simulink library "sm_wheel_loader_lib"  (R2025a)
settings: Solver=VariableStepAuto  StartTime=0.0  StopTime=10.0  RelTol=1e-3
undefined symbols (not defined in the file): AToTOrificeVector, BiPOrificeVector, boomHEArea, boomREArea, BToTOrificeVector, fluids, GRake, GToothL, GToothR, HMPST, HydFcnParams, logLoad, Position, PToAOrificeVector, PToBOrificeVector, RakeL, RakeR, testInput, Wheel_Loader, X, Y, Z
libraries: sm_lib x694, fl_lib x183, nesl_utility x74, SimscapeFluids_lib x62, sdl_lib x25, cvt_components_lib x25, simulink_extras x5, $bdroot x4, wheel_loader_contact_lib x4, ee_lib x2, SignalEditorBlockLib x1, batteryecm_lib x1
(part 1 of 26)
Description:
  | Copyright 2023-2025 The MathWorks, Inc.
settings Model: VariantFading=off  Creator=smiller  LastModifiedBy=smiller
settings RTWCC: GPUComputeCapability=3.5

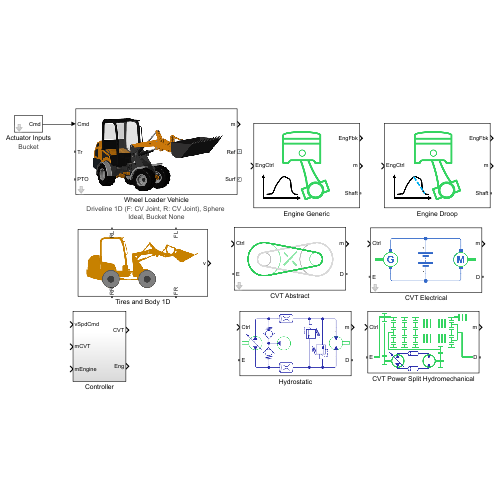
[thumbnail: Simulink's stored preview of the top-level diagram]
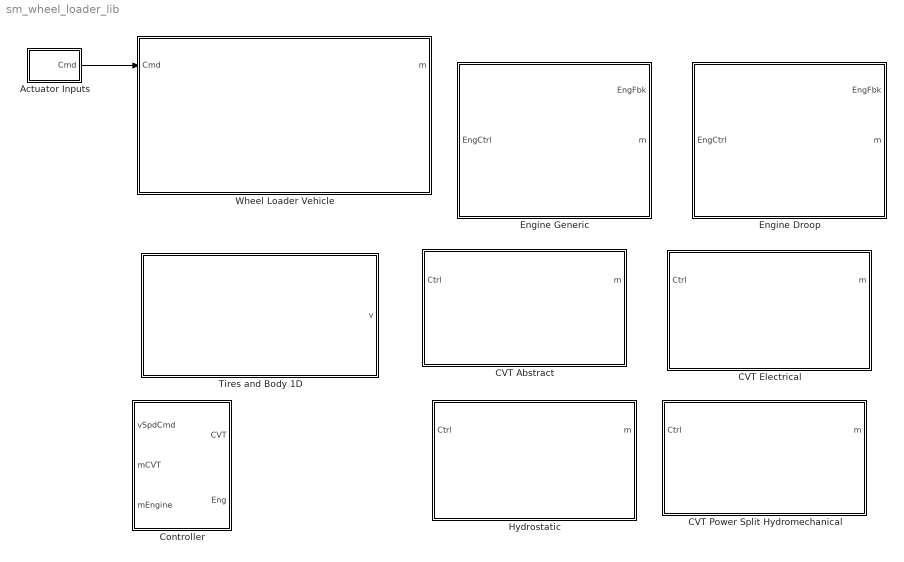
== system sm_wheel_loader_lib ==
  Actuator Inputs : Subsystem  mask{popup_steering=on, popup_linkage=on, popup_impl=Bucket}
      mask prompts: popup_steering "Enable Steering"; popup_linkage "Enable Linkage"; popup_impl "Implement"
      mask init:
      | if(popup_steering)
      |     set_param([gcb '/Enable Steering'],'Gain','1')
      | else
      |     set_param([gcb '/Enable Steering'],'Gain','0')
      | end
      | if(popup_linkage)
      |     set_param([gcb '/Enable Linkage'],'Gain','1')
      | else
      |     set_param([gcb '/Enable Linkage'],'Gain','0')
      | end
      | 
      | if(strcmp(get_param(gcb,'popup_impl'),'Grapple'))
      |     set_param([gcb '/Signal Editor'],'ActiveScenario','GrappleLogCycle')
      | else
      |     set_param([gcb '/Signal Editor'],'ActiveScenario','BucketYCycle')
      | end
      settings: AttributesFormatString=%<popup_impl>
      mask TypeOptions popup_impl: Grapple | Bucket
  CVT Abstract : Subsystem  mask(Continuously Variable Transmission (Abstract)){dShaftE=HMPST.AbstractCVT.dInput, dShaftD=HMPST.AbstractCVT.dOutput, k=HMPST.AbstractCVT.kCompliance, d=HMPST.AbstractCVT.dCompliance}
      mask prompts: dShaftE "Damping Engine Shaft (N*m/(rad/s))"; dShaftD "Damping Driveline Shaft (N*m/(rad/s))"; k "Compliance Stiffness (N*m/rad)"; d "Compliance Damping (N*m/(rad/s))"
      mask help: Models a CVT as a variable ratio gear. The ratio can be negative, positive, or zero. Separate damping elements are connected to the input and output shafts to represent viscous friction. A small compliant element captures dynamics within the transmission.
      mask TypeOptions dShaftE:
      | Variable
      | Gear Box/dInput
      mask TypeOptions dShaftD:
      | Variable
      | Gear Box/dOutput
      mask TypeOptions k:
      | Variable
      | Gear Box/k
      mask TypeOptions d:
      | Variable
      | Gear Box/d
      mask Display: image('ssc_cvt_abstract_IMAGE.png')
  CVT Electrical : Subsystem  VariantControl=Electrical  mask(Electrical Continuously Variable Transmission (eCVT)){}
      mask help:
      | Models a CVT using a generator, motor, and a battery.
      |
      | The input shaft drives a generator which is electrically connected to a motor which mechanically connected to the drivetrain.  A control system adjusts the torque request to the generator and motor so that the desired ratio of (input shaft speed/output shaft speed) is achieved.
      |
      | The power source on the DC bus maintains stability of the DC bus and provides the current required of the motor that the generator cannot provide.  This can be due to variations in time constants for the motor and generator or if the generator reaches its power limit.
      mask Display: image('ssc_electrical_cvt_IMAGE.png')
  CVT Power Split Hydromechanical : Subsystem
      mask Display: image('ssc_hydromech_power_split_cvt_IMAGE.png');
  Controller : Subsystem
  Engine Droop : Subsystem  VariantControl=Droop
      mask Display: image('sdl_engine_Droop_IMAGE.png')
  Engine Generic : Subsystem  VariantControl=Generic
      mask Display: image('sdl_engine_Generic_IMAGE.png');
  Hydrostatic : Subsystem  VariantControl=Hydrostatic
      mask Display: image('sm_wheel_loader_hydrostatic_IMAGE.png');
  Tires and Body 1D : Subsystem
      settings: PortSchema="{\"entries\":[{\"content\":{\"sides\":[{\"content\":{\"connectorIds\":[\"LConn1\",\"LConn2\"]},\"type\":\"ConnectorPlacement.EquallySpacedRectSide\",\"uuid\":\"f6e4eca3-fb02-4523-87a7-c8328825f67f\"},{\"content\":{\"connectorIds\":[\"RConn1\",\"RConn2\"],\"side\":\"RIGHT\"},\"type\":\"ConnectorPlacement.EquallySpacedRectSide\",\"uuid\":\"a01e7d42-3992-448e-add1-f2755d8f064c\"},{\"content\":{\"connectorIds\":[\"Out1\"],\"side\":\"TOP\"},\"type\":\"ConnectorPlacement.EquallySpacedRectSide\",\"uuid\":\"cf483cf6-51ef-4c82-b2ec-fd42745a5c51\"},{\"content\":{\"side\":\"BOTTOM\"},\"type\":\"ConnectorPlacement.EquallySpacedRectSide\",\"uuid\":\"9bbb772c-3b9f-4e30-8c40-373d820ff5eb\"}]},\"type\":\"ConnectorPlacement.EquallySpacedConnector\",\"uuid\":\"52398d34-f462-4e1c-abff-1dda3b221c82\"}],\"packageUris\":[\"http://schema.mathworks.com/mf0/Connector/R2020b\"],\"version\":\"1.0\"}"
      mask Display: image('sm_wheel_loader_vehicle1D_Rot_IMAGE.png');
  Wheel Loader Vehicle : Subsystem  VariantControl=simVariant == 1  mask(Wheel Loader Vehicle){popup_impl=Bucket, popup_actuator_model=Ideal, popup_load=None, popup_driveline_model=Driveline 1D, popup_driveJointF=CV Joint, popup_driveJointR=CV Joint, popup_contact=Sphere}
      mask prompts: popup_impl "Implement"; popup_actuator_model "Actuator Model"; popup_load "Load"; popup_driveline_model "Driveline Model"; popup_driveJointF "Driveline Joint (front)"; popup_driveJointR "Driveline Joint (rear)"; popup_contact "Contact Geometry"
      mask help: Models chassis, driveline, and linkage for a wheel loader. Use drop down menus to configure system options.
      mask init:
      | set_param([gcb '/Load'],'LabelModeActiveChoice',get_param(gcb,'popup_load'));
      | if(strcmp(get_param(gcb,'popup_driveline_model'),'Driveline 3D'))
      |     set_param([gcb '/Driveline'],'popup_driveJointF',...
      |         get_param(gcb,'popup_driveJointF'));
      |     set_param([gcb '/Driveline'],'popup_driveJointR',...
      |         get_param(gcb,'popup_driveJointR'));
      |     
      | end
      | if(strcmp(get_param(gcb,'popup_actuator_model'),'Ideal'))
      |     set_param([gcb '/Actuators'],'LabelModeActiveChoice','Ideal');
      |     set_param([gcb '/Steering Actuator'],'popup_actuator_model','Position');
      |     set_param([gcb '/Linkage'],'popup_actuator_model','Position');
      | elseif(strcmp(get_param(gcb,'popup_actuator_model'),'Hydraulic'))
      |     set_param([gcb '/Actuators'],'LabelModeActiveChoice','Hydraulic');
      |     set_param([gcb '/Steering Actuator'],'popup_actuator_model','Shaft');
      |     set_param([gcb '/Linkage'],'popup_actuator_model','Shaft');
      | end
      settings: AttributesFormatString=|
      | %<popup_driveline_model> (F: %<popup_driveJointF>, R: %<popup_driveJointR>), %<popup_contact>
      | %<popup_actuator_model>, %<popup_impl> %<popup_load>
      mask TypeOptions popup_impl: Actuators/popup_impl | Linkage/popup_impl
      mask TypeOptions popup_actuator_model: Ideal | Hydraulic
      mask TypeOptions popup_load: None | Log | Inertia
      mask TypeOptions popup_driveline_model: Driveline/popup_driveline_model
      mask Callback popup_driveline_model: maskObj = Simulink.Mask.get(gcb);
      mask TypeOptions popup_driveJointF: CV Joint | U Joint
      mask TypeOptions popup_driveJointR: CV Joint | U Joint
      mask TypeOptions popup_contact: Driveline/popup_contact
      mask Display: image('sm_wheel_loader_vehicle_IMAGE.png');
  wires:
  Actuator Inputs/1(Cmd) -> Wheel Loader Vehicle/1(Cmd)

== system sm_wheel_loader_lib/Actuator Inputs ==
  Bus Creator{,1..4} (5 alike) : BusCreator  Inputs=1
  Bus Creator5 : BusCreator  Inputs=6
  Bus Creator6 : BusCreator  Inputs=5
  Bus Creator7 : BusCreator  Inputs=2
  Clock : Clock
  Enable Linkage : Gain
  Enable Steering : Gain
  Inertia Bucket : Lookup_n-D  NumberOfTableDimensions=1  BreakpointsForDimension1=testInput.Active.bucketLoad.t  Table=testInput.Active.bucketLoad.z  InternalRulePriority=Speed  RndMeth=Simplest
  Lift : Lookup_n-D  NumberOfTableDimensions=1  BreakpointsForDimension1=testInput.Active.Lift.t  Table=testInput.Active.Lift.p*1000  InterpMethod=Cubic spline  InternalRulePriority=Speed  RndMeth=Simplest
  Signal Editor : SignalEditorBlockLib/Signal Editor  FileName=sm_wheel_loader_test_operator_cmd.mat  ActiveScenario=BucketYCycle  ActiveSignal=vVehPcnt  IsBus=off  OutputBusObjectStr=Bus: BusObject  SampleTime=0  ZeroCross=off  OutputAfterFinalValue=Setting to zero  Unit=inherit  PreserveSignalName=on  ApplySigPropsToAllScenarios=on  ApplySigPropsToAllSignals=off  SignalPropertySource=Dialog parameters
  Steer : Lookup_n-D  NumberOfTableDimensions=1  BreakpointsForDimension1=testInput.Active.Steer.t  Table=testInput.Active.Steer.p*1000  InterpMethod=Akima spline  InternalRulePriority=Speed  RndMeth=Simplest
  Tilt : Lookup_n-D  NumberOfTableDimensions=1  BreakpointsForDimension1=testInput.Active.Tilt.t  Table=testInput.Active.Tilt.p*1000  InterpMethod=Cubic spline  InternalRulePriority=Speed  RndMeth=Simplest
  Toothbar : Lookup_n-D  NumberOfTableDimensions=1  BreakpointsForDimension1=testInput.Active.Toothbar.t  Table=testInput.Active.Toothbar.p  InternalRulePriority=Speed  RndMeth=Simplest
  Cmd : Outport
  wires:
  Enable Linkage/1 -> Toothbar/1, Tilt/1, Lift/1
  Bus Creator4/1 -> Bus Creator5/5  "rightToothbarAct"
  Bus Creator/1 -> Bus Creator5/1  "steeringAct"
  Steer/1 -> Bus Creator/1  "pos"
  Bus Creator2/1 -> Bus Creator5/3  "tiltAct"
  Clock/1 -> Inertia Bucket/1, Enable Linkage/1, Enable Steering/1
  Bus Creator3/1 -> Bus Creator5/4  "leftToothbarAct"
  Toothbar/1 -> Bus Creator4/1, Bus Creator3/1  "pos"
  Bus Creator1/1 -> Bus Creator5/2  "liftAct"
  Bus Creator5/1 -> Bus Creator7/1  "Actuator"
  Enable Steering/1 -> Steer/1
  Tilt/1 -> Bus Creator2/1  "pos"
  Lift/1 -> Bus Creator1/1  "pos"
  Inertia Bucket/1 -> Bus Creator5/6  "InertiaLoad"
  Signal Editor/1 -> Bus Creator6/1
  Signal Editor/2 -> Bus Creator6/2
  Signal Editor/3 -> Bus Creator6/3
  Bus Creator6/1 -> Bus Creator7/2  "Operator"
  Bus Creator7/1 -> Cmd/1
  Signal Editor/4 -> Bus Creator6/4
  Signal Editor/5 -> Bus Creator6/5

== system sm_wheel_loader_lib/CVT Abstract ==
  BusElementIn1 : Inport  PortName=Ctrl  Element=ratio
  BusElementIn2 : Inport  PortName=Ctrl  Element=CmdVehSpdDir
  Bearing Friction : sdl_lib/Couplings & Drives/Springs & Dampers/Rotational Damper  D=HMPST.Bearing.dVisc N*m*s/rad  thermal_port=simscape.enum.thermaleffects.omit  thermal_mass=50 kJ/K  temperature_specify=off  temperature_priority=High  temperature=300 K  temperature_nominal_specify=off  temperature_nominal_value=1  temperature_nominal_unit=K
  Constant : Constant  Value=0
  Mechanical Rotational Reference : fl_lib/Mechanical/Rotational Elements/Mechanical Rotational Reference
  Product : Product
  Sensor wIn : Subsystem
  Sensor wOut : Subsystem
  Simulink-PS Converter : nesl_utility/Simulink-PS Converter  PhysicalDomain=network_engine_domain  SubClassName=ps_input  LeftPortType=input  RightPortType=output  PseudoPeriodic=off  Frequencies=[]  NoiseDistribution=none  NoiseParameters=[]  Unit=1  AffineConversion=off  FilteringAndDerivatives=provide  SimscapeFilterOrder=1  InputFilterTimeConstant=0.001  UdotUserProvided=0
  Variable Gear Box : cvt_components_lib/Variable Gear Box  k=k  d=d  dInput=dShaftE  dOutput=dShaftD
  E : PMIOPort  Side=Left
  D : PMIOPort  Port=2  Side=Right
  Out Bus Element : Outport  PortName=m  Element=wIn
  Out Bus Element11 : Outport  PortName=m  Element=OutputShaft
  Out Bus Element12 : Outport  PortName=m  Element=P_acc
  wires:
  Product/1 -> Simulink-PS Converter/1
  Constant/1 -> Out Bus Element12/1  "P_acc"
  Sensor wOut/1(w) -> Out Bus Element11/1
  Sensor wIn/1(w) -> Out Bus Element/1
  BusElementIn2/1 -> Product/2
  BusElementIn1/1 -> Product/1
  connections:
  Variable Gear Box/LConn2 -- Sensor wIn/LConn1 -- E/RConn1
  Simulink-PS Converter/RConn1 -- Variable Gear Box/LConn1
  D/RConn1 -- Bearing Friction/LConn1 -- Sensor wOut/LConn1 -- Variable Gear Box/RConn1
  Bearing Friction/RConn1 -- Mechanical Rotational Reference/LConn1

== system sm_wheel_loader_lib/CVT Electrical ==
  BusElementIn1 : Inport  PortName=Ctrl  Element=ratio
  BusElementIn2 : Inport  PortName=Ctrl  Element=CmdVehSpdDir
  Battery : batteryecm_lib/Battery  Vnom=HMPST.eCVT.Battery.Vnom V  prm_dir=simscape.enum.battery.prm_dir.disabled  R1_dis=2 Ohm  R1_ch=2 Ohm  R1=HMPST.eCVT.Battery.Rint Ohm  prm_AH=simscape.enum.battery.prm_AH.finite  AH=HMPST.eCVT.Battery.AH A*hr  V1=HMPST.eCVT.Battery.V1 V  AH1=HMPST.eCVT.Battery.AH1 A*hr  prm_R2=simscape.enum.battery.prm_R2.disabled  R2=2000 Ohm  Tmeas=298.15 K  charge_measurement_port=simscape.enum.battery.enable.no  prm_dyn=simscape.enum.battery.prm_dyn.off  Rp1=0.005 Ohm  tau1=30 s  Rp2=0.005 Ohm  tau2=30 s  Rp3=0.005 Ohm  tau3=30 s  Rp4=0.005 Ohm  tau4=30 s  Rp5=0.005 Ohm  tau5=30 s  prm_fade=simscape.enum.battery.prm_fade.disabled  N_fade=100  AH_fade=45 A*hr  R1_fade=2.02 Ohm  R1_ch_fade=2.02 Ohm  V1_fade=10.35 V  prm_age=simscape.enum.battery.prm_age.disabled  prm_age_OCV=simscape.enum.battery.prm_age_OCV.OCV  OCV_age=0.9  SOC_age=60  Tmeas_age=298.15 K  delta_time_age_vec=[0] d  temperature_age_vec=[273] K  OCV_scaling_age=2.2134e6  OCV_offset_age=1.632e6  temp_exp_age=0.515833569 V  t_exp_age=0.75  Vnom_T2=12 V  R1_T2=2.2 Ohm  R1_T2_dis=2.2 Ohm  R1_T2_ch=2.2 Ohm  V1_T2=11.4 V  R2_T2=2200 Ohm  Rp1_T2=0.005 Ohm  tau1_T2=30 s  Rp2_T2=0.005 Ohm  tau2_T2=30 s  Rp3_T2=0.005 Ohm  tau3_T2=30 s  Rp4_T2=0.005 Ohm  tau4_T2=30 s  Rp5_T2=0.005 Ohm  tau5_T2=30 s  Tmeas2=273.15 K  thermal_port=simscape.enum.thermaleffects.omit  thermal_mass=30000 J/K  i_specify=off  i_priority=None  i=0 A  i_nominal_specify=off  i_nominal_value=1  i_nominal_unit=A  v_specify=off  v_priority=None  v=0 V  v_nominal_specify=off  v_nominal_value=1  v_nominal_unit=V  charge_specify=on  charge_priority=High  charge=HMPST.eCVT.Battery.AH A*hr  charge_nominal_specify=off  charge_nominal_value=1  charge_nominal_unit=A*hr  num_cycles_specify=off  num_cycles_priority=High  num_cycles=0  num_cycles_nominal_specify=off  num_cycles_nominal_value=1  num_cycles_nominal_unit=1  temperature_specify=off  temperature_priority=High  temperature=298.15 K  temperature_nominal_specify=off  temperature_nominal_value=1  temperature_nominal_unit=K
  Constant : Constant  Value=0
  Control : Subsystem
  Electrical Reference : fl_lib/Electrical/Electrical Elements/Electrical Reference
  Gear Box : fl_lib/Mechanical/Mechanisms/Gear Box  ratio=-1  t_in_specify=off  t_in_priority=None  t_in=0 N*m  t_in_nominal_specify=off  t_in_nominal_value=1  t_in_nominal_unit=N*m  t_out_specify=off  t_out_priority=None  t_out=0 N*m  t_out_nominal_specify=off  t_out_nominal_value=1  t_out_nominal_unit=N*m
  Generator : ee_lib/Electromechanical/Motor & Drive (System Level)  torque_speed_param=ee.enum.electromech.envelope.tabulated  overtorque_param=ee.enum.electromech.overtorque.no  T_t=HMPST.eCVT.Generator.trqSpd.t N*m  T_t_intermittent=[.36, .32, .28, 0] N*m  T_t_2D=[.09, .09, .09; .08, .08, .08; .07, .07, .07; 0, 0, 0] N*m  T_t_intermittent_2D=[.36, .36, .36; .32, .32, .32; .28, .28, .28; 0, 0, 0] N*m  w_t=HMPST.eCVT.Generator.trqSpd.w rpm  vdc_t=[6, 12, 24] V  torque_max=0.1 N*m  power_max=30 W  torque_max_intermittent=0.4 N*m  power_max_intermittent=120 W  time_overtorque=30 s  time_recover=60 s  Tc=HMPST.eCVT.Generator.Tc s  EnableSwitch=simscape.enum.onoff.off  losses_param=1  eff=100  w_eff=3750 rpm  T_eff=0.08 N*m  Piron=0 W  Pbase=0 W  w_eff_vec=[-8000, -4000, 0, 4000, 8000] rpm  T_eff_vec=[0, .03, .06, .09] N*m  v_eff_vec=[100, 250, 400] V  losses_mat=[1.49, 1.67, 2.21, 3.1; .42, .69, 1.14, 2.03; .06, .24, .78, 1.68; .42, .69, 1.14, 2.03; 1.49, 1.67, 2.21, 3.1] W  efficiency_mat=[95, 95, 95, 95; 95, 95, 95, 95; 95, 95, 95, 95; 95, 95, 95, 95; 95, 95, 95, 95]  losses_mat_3D=ones(5, 4, 3) W  efficiency_mat_3D=95 * ones(5, 4, 3)  Res=0 Ohm  J=HMPST.eCVT.Generator.J kg*m^2  lam=HMPST.eCVT.Generator.lam N*m*s/rad  speed0=HMPST.eCVT.Generator.w0 rpm  faulted_specify=off  faulted_priority=None  faulted=0  faulted_nominal_specify=off  faulted_nominal_value=1  faulted_nominal_unit=1  isSwitchedOff_specify=off  isSwitchedOff_priority=None  isSwitchedOff=0  isSwitchedOff_nominal_specify=off  isSwitchedOff_nominal_value=1  isSwitchedOff_nominal_unit=1  torqueLimitContinuous_specify=off  torqueLimitContinuous_priority=None  torqueLimitContinuous=0 N*m  torqueLimitContinuous_nominal_specify=off  torqueLimitContinuous_nominal_value=1  torqueLimitContinuous_nominal_unit=N*m  alpha=3.93e-3 1/K  Tmeas=25 degC  Tmeas2=125 degC  losses_mat_T2=[1.49, 1.74, 2.49, 3.74; .42, .67, 1.42, 2.67; .06, .31, 1.06, 2.31; .42, .67, 1.42, 2.67; 1.49, 1.74, 2.49, 3.74] W  efficiency_mat_T2=[95, 95, 95, 95; 95, 95, 95, 95; 95, 95, 95, 95; 95, 95, 95, 95; 95, 95, 95, 95]  losses_mat_3D_T2=ones(5, 4, 3) W  efficiency_mat_3D_T2=95 * ones(5, 4, 3)  thermal_mass=100 J/K  initial_temperature=25 degC
  Mechanical Rotational Reference : fl_lib/Mechanical/Rotational Elements/Mechanical Rotational Reference
  Mechanical Rotational Reference1 : fl_lib/Mechanical/Rotational Elements/Mechanical Rotational Reference
  Motor : ee_lib/Electromechanical/Motor & Drive (System Level)  torque_speed_param=ee.enum.electromech.envelope.tabulated  overtorque_param=ee.enum.electromech.overtorque.no  T_t=HMPST.eCVT.Motor.trqSpd.t N*m  T_t_intermittent=[.36, .32, .28, 0] N*m  T_t_2D=[.09, .09, .09; .08, .08, .08; .07, .07, .07; 0, 0, 0] N*m  T_t_intermittent_2D=[.36, .36, .36; .32, .32, .32; .28, .28, .28; 0, 0, 0] N*m  w_t=HMPST.eCVT.Motor.trqSpd.w rpm  vdc_t=[6, 12, 24] V  torque_max=0.1 N*m  power_max=30 W  torque_max_intermittent=0.4 N*m  power_max_intermittent=120 W  time_overtorque=30 s  time_recover=60 s  Tc=HMPST.eCVT.Motor.Tc s  EnableSwitch=simscape.enum.onoff.off  losses_param=1  eff=100  w_eff=3750 rpm  T_eff=0.08 N*m  Piron=0 W  Pbase=0 W  w_eff_vec=[-8000, -4000, 0, 4000, 8000] rpm  T_eff_vec=[0, .03, .06, .09] N*m  v_eff_vec=[100, 250, 400] V  losses_mat=[1.49, 1.67, 2.21, 3.1; .42, .69, 1.14, 2.03; .06, .24, .78, 1.68; .42, .69, 1.14, 2.03; 1.49, 1.67, 2.21, 3.1] W  efficiency_mat=[95, 95, 95, 95; 95, 95, 95, 95; 95, 95, 95, 95; 95, 95, 95, 95; 95, 95, 95, 95]  losses_mat_3D=ones(5, 4, 3) W  efficiency_mat_3D=95 * ones(5, 4, 3)  Res=0 Ohm  J=HMPST.eCVT.Motor.J kg*m^2  lam=HMPST.eCVT.Motor.lam N*m*s/rad  speed0=HMPST.eCVT.Motor.w0 rpm  faulted_specify=off  faulted_priority=None  faulted=0  faulted_nominal_specify=off  faulted_nominal_value=1  faulted_nominal_unit=1  isSwitchedOff_specify=off  isSwitchedOff_priority=None  isSwitchedOff=0  isSwitchedOff_nominal_specify=off  isSwitchedOff_nominal_value=1  isSwitchedOff_nominal_unit=1  torqueLimitContinuous_specify=off  torqueLimitContinuous_priority=None  torqueLimitContinuous=0 N*m  torqueLimitContinuous_nominal_specify=off  torqueLimitContinuous_nominal_value=1  torqueLimitContinuous_nominal_unit=N*m  alpha=3.93e-3 1/K  Tmeas=25 degC  Tmeas2=125 degC  losses_mat_T2=[1.49, 1.74, 2.49, 3.74; .42, .67, 1.42, 2.67; .06, .31, 1.06, 2.31; .42, .67, 1.42, 2.67; 1.49, 1.74, 2.49, 3.74] W  efficiency_mat_T2=[95, 95, 95, 95; 95, 95, 95, 95; 95, 95, 95, 95; 95, 95, 95, 95; 95, 95, 95, 95]  losses_mat_3D_T2=ones(5, 4, 3) W  efficiency_mat_3D_T2=95 * ones(5, 4, 3)  thermal_mass=100 J/K  initial_temperature=25 degC
  PS-Simulink Converter2 : nesl_utility/PS-Simulink Converter  PhysicalDomain=network_engine_domain  SubClassName=ps_output  LeftPortType=input  RightPortType=output  PseudoPeriodic=off  Frequencies=[]  VectorFormat=inherit  Unit=rpm  AffineConversion=off
  PS-Simulink Converter3 : nesl_utility/PS-Simulink Converter  PhysicalDomain=network_engine_domain  SubClassName=ps_output  LeftPortType=input  RightPortType=output  PseudoPeriodic=off  Frequencies=[]  VectorFormat=inherit  Unit=rpm  AffineConversion=off
  Product2 : Product
  Simulink-PS Converter1 : nesl_utility/Simulink-PS Converter  PhysicalDomain=network_engine_domain  SubClassName=ps_input  LeftPortType=input  RightPortType=output  PseudoPeriodic=off  Frequencies=[]  NoiseDistribution=none  NoiseParameters=[]  Unit=1  AffineConversion=off  FilteringAndDerivatives=provide  SimscapeFilterOrder=1  InputFilterTimeConstant=0.001  UdotUserProvided=0
  Simulink-PS Converter2 : nesl_utility/Simulink-PS Converter  PhysicalDomain=network_engine_domain  SubClassName=ps_input  LeftPortType=input  RightPortType=output  PseudoPeriodic=off  Frequencies=[]  NoiseDistribution=none  NoiseParameters=[]  Unit=1  AffineConversion=off  FilteringAndDerivatives=provide  SimscapeFilterOrder=1  InputFilterTimeConstant=0.001  UdotUserProvided=0
  E : PMIOPort  Side=Left
  D : PMIOPort  Port=2  Side=Right
  Out Bus Element11 : Outport  PortName=m  Element=OutputShaft
  Out Bus Element12 : Outport  PortName=m  Element=P_acc
  Out Bus Element1 : Outport  PortName=m  Element=wIn
  wires:
  BusElementIn1/1 -> Product2/1
  BusElementIn2/1 -> Product2/2
  Constant/1 -> Out Bus Element12/1  "P_acc"
  PS-Simulink Converter2/1 -> Out Bus Element11/1, [wOut]
  Product2/1 -> Control/1(ratioCmd)
  [wOut] -> Control/2(wOut)
  [wIn] -> Control/3(wIn)
  Control/2(trqGen) -> Simulink-PS Converter2/1
  Control/1(trqMot) -> Simulink-PS Converter1/1
  PS-Simulink Converter3/1 -> [wIn], Out Bus Element1/1
  connections:
  Motor/LConn3 -- Gear Box/LConn1
  E/RConn1 -- Generator/LConn3
  PS-Simulink Converter2/LConn1 -- Motor/RConn2
  Electrical Reference/LConn1 -- Battery/RConn1 -- Motor/RConn1 -- Generator/RConn1
  Simulink-PS Converter1/RConn1 -- Motor/LConn2
  Generator/RConn3 -- Mechanical Rotational Reference/LConn1
  Motor/RConn3 -- Mechanical Rotational Reference1/LConn1
  Simulink-PS Converter2/RConn1 -- Generator/LConn2
  PS-Simulink Converter3/LConn1 -- Generator/RConn2
  Motor/LConn1 -- Generator/LConn1 -- Battery/LConn1
  Gear Box/RConn1 -- D/RConn1

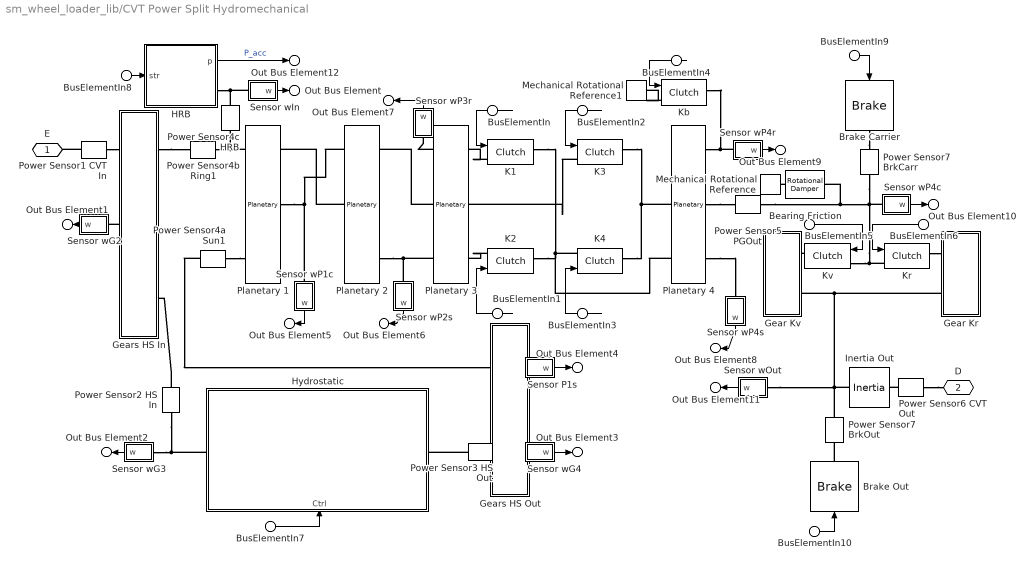
== system sm_wheel_loader_lib/CVT Power Split Hydromechanical ==
  BusElementIn : Inport  PortName=Ctrl  Element=K1
  BusElementIn1 : Inport  PortName=Ctrl  Element=K2
  BusElementIn2 : Inport  PortName=Ctrl  Element=K3
  BusElementIn3 : Inport  PortName=Ctrl  Element=K4
  BusElementIn4 : Inport  PortName=Ctrl  Element=Kb
  BusElementIn5 : Inport  PortName=Ctrl  Element=Kv
  BusElementIn6 : Inport  PortName=Ctrl  Element=Kr
  BusElementIn7 : Inport  PortName=Ctrl  Element=SwashCtrl
  BusElementIn8 : Inport  PortName=Ctrl  Element=HRBCtrl
  BusElementIn9 : Inport  PortName=Ctrl  Element=MBCtrl
  BusElementIn10 : Inport  PortName=Ctrl  Element=MBCtrl
  Bearing Friction : sdl_lib/Couplings & Drives/Springs & Dampers/Rotational Damper  D=HMPST.Bearing.dVisc N*m*s/rad  thermal_port=simscape.enum.thermaleffects.omit  thermal_mass=50 kJ/K  temperature_specify=off  temperature_priority=High  temperature=300 K  temperature_nominal_specify=off  temperature_nominal_value=1  temperature_nominal_unit=K
  Brake Carrier : cvt_components_lib/Brake  bore=HMPST.Brake.cylBore  brkwy_vel=HMPST.Brake.vBrk  mu_static=HMPST.Brake.muSta  mu_coulomb=HMPST.Brake.muKin  n_pads=HMPST.Brake.numPads  r_mean=HMPST.Brake.rPad  visc_coef=HMPST.Brake.dVisc  logic2pressure=HMPST.Brake.logic2Press  ts_filt=HMPST.Brake.tsFilt
  Brake Out : cvt_components_lib/Brake  bore=HMPST.Brake.cylBore  brkwy_vel=HMPST.Brake.vBrk  mu_static=HMPST.Brake.muSta  mu_coulomb=HMPST.Brake.muKin  n_pads=HMPST.Brake.numPads  r_mean=HMPST.Brake.rPad  visc_coef=HMPST.Brake.dVisc  logic2pressure=HMPST.Brake.logic2Press  ts_filt=HMPST.Brake.tsFilt
  Gear Kr : Subsystem
      mask Display: image('sm_wheel_loader_CVTGOut_IMAGE.png');
  Gear Kv : Subsystem
      mask Display: image('sm_wheel_loader_CVTGOut_IMAGE.png');
  Gears HS In : Subsystem
      mask Display: image('sm_wheel_loader_HSGIn_IMAGE.png')
  Gears HS Out : Subsystem
      mask Display: image('sm_wheel_loader_HSGOut_IMAGE.png');
  HRB : Subsystem
      mask Display: image('sm_wheel_loader_HRB_IMAGE.png');
  Hydrostatic : Subsystem  mask(Hydrostatic Transmission){pumpNomDisp=HMPST.HydroUnit.Pump.Disp, motorNomDisp=HMPST.HydroUnit.Motor.Disp, pumpNomSpd=HMPST.HydroUnit.Pump.SpeedLimit, motorNomSpd=HMPST.HydroUnit.Motor.wNominal, pumpNomVolEff=HMPST.HydroUnit.Pump.volEffNominal, motorNomVolEff=HMPST.HydroUnit.Motor.volEffNominal, pumpNomMechEff=HMPST.HydroUnit.Pump.mechEffNominal, motorNomMechEff=HMPST.HydroUnit.Motor.mechEffNominal, pumpNomPressGain=HMPST.HydroUnit.Pump.prGainNominal, motorNomPressDrop=HMPST.HydroUnit.Motor.prDropNominal, p_crack_differential=HMPST.HydroUnit.ChkV.pDiffCrack, press_max_differential=HMPST.HydroUnit.ChkV.pDiffMax, chkv_area_max=HMPST.HydroUnit.ChkV.aMax, chkv_area_leak=HMPST.HydroUnit.ChkV.aLeak, p_set_differential=HMPST.HydroUnit.PrV.pDiffSet, p_range=HMPST.HydroUnit.PrV.pRange, prv_area_max=HMPST.HydroUnit.PrV.aMax, prv_area_leak=HMPST.HydroUnit.PrV.aLeak, pipeLen=HMPST.HydroUnit.Pipes.len, pipeAreaGeo=HMPST.HydroUnit.Pipes.aGeom, pipeAreaHydr=HMPST.HydroUnit.Pipes.aHydr, chgPumpNomDisp=HMPST.HydroUnit.ChargePump.Disp, chgPumpNomMechEff=HMPST.HydroUnit.ChargePump.mechEffNominal, chgPumpNomPressGain=HMPST.HydroUnit.ChargePump.prGainNominal, chgPumpNomSpd=HMPST.HydroUnit.ChargePump.wNominal, chgPumpNomVolEff=HMPST.HydroUnit.ChargePump.volEffNominal, chgPumpChkvAleak=HMPST.HydroUnit.ChargePumpPrV.aLeak, chgPumpChkvAmax=HMPST.HydroUnit.ChargePumpPrV.aMax, chgPumpChkvPdiff=HMPST.HydroUnit.ChargePumpPrV.pDiffSet, chgPumpChkvPrange=HMPST.HydroUnit.ChargePumpPrV.pRange}
      mask prompts: pumpNomDisp "Pump Nominal Disp. (cm^3/rev)"; motorNomDisp "Motor Nominal Disp. (cm^3/rev)"; pumpNomSpd "Pump Nominal Speed (rpm)"; motorNomSpd "Motor Nominal Speed (rpm)"; pumpNomVolEff "Pump Nominal Volumentric Eff. (0-1)"; motorNomVolEff "Motor Nominal Volumentric Eff. (0-1)"; pumpNomMechEff "Pump Nominal Mechanical Eff. (0-1)"; motorNomMechEff "Motor Nominal Mechanical Eff. (0-1)"; pumpNomPressGain "Pump Nominal Pressure Gain (MPa)"; motorNomPressDrop "Motor Nominal Pressure Drop (MPa)"; p_crack_differential "Cracking pressure differential (MPa)"; press_max_differential "Maximum opening pressure differential (MPa)"; chkv_area_max "Maximum opening area (m^2)"; chkv_area_leak "Leakage area (m^2)"; p_set_differential "Set pressure differential"; p_range "Pressure regulation range"; prv_area_max "Maximum opening area"; prv_area_leak "Leakage area"; pipeLen "Pipe length (m)"; pipeAreaGeo "Cross-sectional area (m^2)"; pipeAreaHydr "Hydraulic diameter (m^2)"; chgPumpNomDisp "Displacement (cm^3/rev)"; chgPumpNomMechEff "Nominal Mechanical Efficiency (0-1)"; chgPumpNomPressGain "Nominal pressure gain (MPa)"; chgPumpNomSpd "Nominal Angular Velocity (rpm)"; chgPumpNomVolEff "Nominal Volumetric Efficiency (0-1)"; chgPumpChkvAleak "Leakage area (m^2)"; chgPumpChkvAmax "Maximum opening area (m^2)"; chgPumpChkvPdiff "Set pressure differential (MPa)"; chgPumpChkvPrange "Pressure regulation range (MPa)"
      mask help: Models a hydrostatic transmission with variable-displacement pump and fixed-displacement motor.
      settings: PortSchema="{\"entries\":[{\"content\":{\"sides\":[{\"content\":{\"connectorIds\":[\"LConn1\"]},\"type\":\"ConnectorPlacement.EquallySpacedRectSide\",\"uuid\":\"eaa3b61f-d017-4906-bbf2-8ecd84d259f8\"},{\"content\":{\"connectorIds\":[\"RConn1\"],\"side\":\"RIGHT\"},\"type\":\"ConnectorPlacement.EquallySpacedRectSide\",\"uuid\":\"0fbcb9a0-a672-4528-9ae6-239f56fc7398\"},{\"content\":{\"side\":\"TOP\"},\"type\":\"ConnectorPlacement.EquallySpacedRectSide\",\"uuid\":\"6ed16286-b13e-4acc-b8af-dca09e2bc3e1\"},{\"content\":{\"connectorIds\":[\"In1\"],\"side\":\"BOTTOM\"},\"type\":\"ConnectorPlacement.EquallySpacedRectSide\",\"uuid\":\"47271b7b-ddb8-4a1d-8fde-8e6a2ea9439a\"}]},\"type\":\"ConnectorPlacement.EquallySpacedConnector\",\"uuid\":\"ac753e2e-3858-4052-8c29-ca92433da3b6\"}],\"packageUris\":[\"http://schema.mathworks.com/mf0/Connector/R2020b\"],\"version\":\"1.0\"}"
      mask TypeOptions p_crack_differential:
      | Check
      | Valve A/p_crack_differential | Check
      | Valve B/p_crack_differential
      mask TypeOptions press_max_differential:
      | Check
      | Valve A/press_max_differential | Check
      | Valve B/press_max_differential
      mask TypeOptions chkv_area_max:
      | Check
      | Valve A/area_max | Check
      | Valve B/area_max
      mask TypeOptions chkv_area_leak:
      | Check
      | Valve A/area_leak | Check
      | Valve B/area_leak
      mask TypeOptions p_set_differential:
      | Pressure
      | Relief
      | Valve A/p_set_differential | Pressure
      | Relief
      | Valve B/p_set_differential
      mask TypeOptions p_range:
      | Pressure
      | Relief
      | Valve A/p_range | Pressure
      | Relief
      | Valve B/p_range
      mask TypeOptions prv_area_max:
      | Pressure
      | Relief
      | Valve A/area_max | Pressure
      | Relief
      | Valve B/area_max
      mask TypeOptions prv_area_leak:
      | Pressure
      | Relief
      | Valve A/area_leak | Pressure
      | Relief
      | Valve B/area_leak
      mask TypeOptions pipeLen: Pipe A /length | Pipe B/length
      mask TypeOptions pipeAreaGeo: Pipe A /area | Pipe B/area
      mask TypeOptions pipeAreaHydr: Pipe A /Dh | Pipe B/Dh
      mask TypeOptions chgPumpNomDisp:
      | Charge
      | Pump/chgPumpNomDisp
      mask TypeOptions chgPumpNomMechEff:
      | Charge
      | Pump/chgPumpNomMechEff
      mask TypeOptions chgPumpNomPressGain:
      | Charge
      | Pump/chgPumpNomPressGain
      mask TypeOptions chgPumpNomSpd:
      | Charge
      | Pump/chgPumpNomSpd
      mask TypeOptions chgPumpNomVolEff:
      | Charge
      | Pump/chgPumpNomVolEff
      mask TypeOptions chgPumpChkvAleak:
      | Charge
      | Pump/chgPumpChkvAleak
      mask TypeOptions chgPumpChkvAmax:
      | Charge
      | Pump/chgPumpChkvAmax
      mask TypeOptions chgPumpChkvPdiff:
      | Charge
      | Pump/chgPumpChkvPdiff
      mask TypeOptions chgPumpChkvPrange:
      | Charge
      | Pump/chgPumpChkvPrange
      mask DialogControl cont_units Prompt: Units
      mask DialogControl cont_valves Prompt: Valves
      mask DialogControl grp_chkv Prompt: Check Valve
      mask DialogControl grp_prv Prompt: Pressure Relief Valve
      mask DialogControl cont_pipes Prompt: Pipes
      mask DialogControl cont_chg_pump Prompt: Charge Pump
      mask DialogControl grp_chg_pump Prompt: Pump
      mask DialogControl grp_chg_pump_prv Prompt: Pressure Relief Valve
      mask Display: image('sm_wheel_loader_hydrostatic_IMAGE.png');
  Inertia Out : fl_lib/Mechanical/Rotational Elements/Inertia  inertia=1 kg*m^2  num_ports=foundation.enum.numPorts2.two  w_specify=off  w_priority=High  w=0 rad/s  w_nominal_specify=off  w_nominal_value=1  w_nominal_unit=rad/s  t_specify=off  t_priority=None  t=0 N*m  t_nominal_specify=off  t_nominal_value=1  t_nominal_unit=N*m
      settings: InternalSimscapePortConfiguration="{\"Bottom\":[],\"Left\":[{\"id\":\"I\",\"label\":\"\",\"type\":\"foundation.mechanical.rotational.rotational\"}],\"Right\":[{\"id\":\"J\",\"label\":\"\",\"type\":\"foundation.mechanical.rotational.rotational\"}],\"Top\":[]}"
  K{1..4} (4 alike) : cvt_components_lib/Clutch  r_eff=HMPST.Clutch.SpdRange.trqRad  nS=HMPST.Clutch.SpdRange.nSurf  piston_area=HMPST.Clutch.SpdRange.aPiston  mu_static=HMPST.Clutch.SpdRange.muSta  mu_coulomb=HMPST.Clutch.SpdRange.muKin  w_tol=HMPST.Clutch.SpdRange.vTol  pressure_min=HMPST.Clutch.SpdRange.pr2Engage  logic_to_pr_gain=HMPST.Clutch.SpdRange.logic2Press  ts_filt=HMPST.Clutch.SpdRange.tsFilt
  Kb : cvt_components_lib/Clutch  r_eff=HMPST.Clutch.SpdRangeBrk.trqRad  nS=HMPST.Clutch.SpdRangeBrk.nSurf  piston_area=HMPST.Clutch.SpdRangeBrk.aPiston  mu_static=HMPST.Clutch.SpdRangeBrk.muSta  mu_coulomb=HMPST.Clutch.SpdRangeBrk.muKin  w_tol=HMPST.Clutch.SpdRangeBrk.vTol  pressure_min=HMPST.Clutch.SpdRangeBrk.pr2Engage  logic_to_pr_gain=HMPST.Clutch.SpdRangeBrk.logic2Press  ts_filt=HMPST.Clutch.SpdRangeBrk.tsFilt
  Kr : cvt_components_lib/Clutch  r_eff=HMPST.Clutch.FwdRev.trqRad  nS=HMPST.Clutch.FwdRev.nSurf  piston_area=HMPST.Clutch.FwdRev.aPiston  mu_static=HMPST.Clutch.FwdRev.muSta  mu_coulomb=HMPST.Clutch.FwdRev.muKin  w_tol=HMPST.Clutch.FwdRev.vTol  pressure_min=HMPST.Clutch.FwdRev.pr2Engage  logic_to_pr_gain=HMPST.Clutch.FwdRev.logic2Press  ts_filt=HMPST.Clutch.FwdRev.tsFilt
  Kv : cvt_components_lib/Clutch  r_eff=HMPST.Clutch.FwdRev.trqRad  nS=HMPST.Clutch.FwdRev.nSurf  piston_area=HMPST.Clutch.FwdRev.aPiston  mu_static=HMPST.Clutch.FwdRev.muSta  mu_coulomb=HMPST.Clutch.FwdRev.muKin  w_tol=HMPST.Clutch.FwdRev.vTol  pressure_min=HMPST.Clutch.FwdRev.pr2Engage  logic_to_pr_gain=HMPST.Clutch.FwdRev.logic2Press  ts_filt=HMPST.Clutch.FwdRev.tsFilt
  Mechanical Rotational Reference : fl_lib/Mechanical/Rotational Elements/Mechanical Rotational Reference
  Mechanical Rotational Reference1 : fl_lib/Mechanical/Rotational Elements/Mechanical Rotational Reference
  Planetary 1 : cvt_components_lib/Planetary  rs_ratio=HMPST.GearTrain.PG1.Ring.TeethNum/HMPST.GearTrain.PG1.Sun.TeethNum  pg_efficiency=[.995, .995]  ring_inertia=0.5  carr_inertia=0.5  sun_inertia=0.5  w_specify=on  w_priority=None  w=0
  Planetary 2 : cvt_components_lib/Planetary  rs_ratio=HMPST.GearTrain.PG2.Ring.TeethNum/HMPST.GearTrain.PG2.Sun.TeethNum  pg_efficiency=[.995, .995]  ring_inertia=0.5  carr_inertia=0.5  sun_inertia=0.5  w_specify=on  w_priority=None  w=0
  Planetary 3 : cvt_components_lib/Planetary  rs_ratio=HMPST.GearTrain.PG3.Ring.TeethNum/HMPST.GearTrain.PG3.Sun.TeethNum  pg_efficiency=[.995, .995]  ring_inertia=0.5  carr_inertia=0.5  sun_inertia=0.5  w_specify=on  w_priority=High  w=0
  Planetary 4 : cvt_components_lib/Planetary  rs_ratio=HMPST.GearTrain.PG4.Ring.TeethNum/HMPST.GearTrain.PG4.Sun.TeethNum  pg_efficiency=[.995, .995]  ring_inertia=0.5  carr_inertia=0.5  sun_inertia=0.5  w_specify=on  w_priority=None  w=0
  Power Sensor1 CVT In : cvt_components_lib/Power Sensor  SystemSampleTime=-1  VariantActivationTime=update diagram  EmptyChoice=off  PassThrough=off  PassThroughVariantControl=(default)  EmptyChoiceVariantControl=(default)  AllowFlexibleInterface=on  Latency=0  AutoFrameSizeCalculation=off
  Power Sensor2 HS In : cvt_components_lib/Power Sensor  SystemSampleTime=-1  VariantActivationTime=update diagram  EmptyChoice=off  PassThrough=off  PassThroughVariantControl=(default)  EmptyChoiceVariantControl=(default)  AllowFlexibleInterface=on  Latency=0  AutoFrameSizeCalculation=off
  Power Sensor3 HS Out : cvt_components_lib/Power Sensor  SystemSampleTime=-1  VariantActivationTime=update diagram  EmptyChoice=off  PassThrough=off  PassThroughVariantControl=(default)  EmptyChoiceVariantControl=(default)  AllowFlexibleInterface=on  Latency=0  AutoFrameSizeCalculation=off
  Power Sensor4a Sun1 : cvt_components_lib/Power Sensor  SystemSampleTime=-1  VariantActivationTime=update diagram  EmptyChoice=off  PassThrough=off  PassThroughVariantControl=(default)  EmptyChoiceVariantControl=(default)  AllowFlexibleInterface=on  Latency=0  AutoFrameSizeCalculation=off
  Power Sensor4b Ring1 : cvt_components_lib/Power Sensor  SystemSampleTime=-1  VariantActivationTime=update diagram  EmptyChoice=off  PassThrough=off  PassThroughVariantControl=(default)  EmptyChoiceVariantControl=(default)  AllowFlexibleInterface=on  Latency=0  AutoFrameSizeCalculation=off
  Power Sensor4c HRB : cvt_components_lib/Power Sensor  SystemSampleTime=-1  VariantActivationTime=update diagram  EmptyChoice=off  PassThrough=off  PassThroughVariantControl=(default)  EmptyChoiceVariantControl=(default)  AllowFlexibleInterface=on  Latency=0  AutoFrameSizeCalculation=off
  Power Sensor5 PGOut : cvt_components_lib/Power Sensor  SystemSampleTime=-1  VariantActivationTime=update diagram  EmptyChoice=off  PassThrough=off  PassThroughVariantControl=(default)  EmptyChoiceVariantControl=(default)  AllowFlexibleInterface=on  Latency=0  AutoFrameSizeCalculation=off
  Power Sensor6 CVT Out : cvt_components_lib/Power Sensor  SystemSampleTime=-1  VariantActivationTime=update diagram  EmptyChoice=off  PassThrough=off  PassThroughVariantControl=(default)  EmptyChoiceVariantControl=(default)  AllowFlexibleInterface=on  Latency=0  AutoFrameSizeCalculation=off
  Power Sensor7 BrkCarr : cvt_components_lib/Power Sensor  SystemSampleTime=-1  VariantActivationTime=update diagram  EmptyChoice=off  PassThrough=off  PassThroughVariantControl=(default)  EmptyChoiceVariantControl=(default)  AllowFlexibleInterface=on  Latency=0  AutoFrameSizeCalculation=off
  Power Sensor7 BrkOut : cvt_components_lib/Power Sensor  SystemSampleTime=-1  VariantActivationTime=update diagram  EmptyChoice=off  PassThrough=off  PassThroughVariantControl=(default)  EmptyChoiceVariantControl=(default)  AllowFlexibleInterface=on  Latency=0  AutoFrameSizeCalculation=off
  Sensor P1s : Subsystem
  Sensor wG2 : Subsystem
  Sensor wG3 : Subsystem
  Sensor wG4 : Subsystem
  Sensor wIn : Subsystem
  Sensor wOut : Subsystem
  Sensor wP1c : Subsystem
  Sensor wP2s : Subsystem
  Sensor wP3r : Subsystem
  Sensor wP4c : Subsystem
  Sensor wP4r : Subsystem
  Sensor wP4s : Subsystem
  E : PMIOPort  Side=Left
  D : PMIOPort  Port=2  Side=Right
  Out Bus Element : Outport  PortName=m  Element=wIn
  Out Bus Element1 : Outport  PortName=m  Element=wG2
  Out Bus Element2 : Outport  PortName=m  Element=wG3_HydIn
  Out Bus Element3 : Outport  PortName=m  Element=wG4_HydOut
  Out Bus Element4 : Outport  PortName=m  Element=wP1s
  Out Bus Element5 : Outport  PortName=m  Element=wP1c
  Out Bus Element6 : Outport  PortName=m  Element=wP2s
  Out Bus Element7 : Outport  PortName=m  Element=wP3r
  Out Bus Element8 : Outport  PortName=m  Element=wP4s
  Out Bus Element9 : Outport  PortName=m  Element=wP4r
  Out Bus Element10 : Outport  PortName=m  Element=wP4c
  Out Bus Element11 : Outport  PortName=m  Element=OutputShaft
  Out Bus Element12 : Outport  PortName=m  Element=P_acc
  wires:
  BusElementIn10/1 -> Brake Out/1
  BusElementIn9/1 -> Brake Carrier/1
  BusElementIn4/1 -> Kb/1
  BusElementIn6/1 -> Kr/1
  BusElementIn5/1 -> Kv/1
  BusElementIn3/1 -> K4/1
  BusElementIn2/1 -> K3/1
  BusElementIn1/1 -> K2/1
  BusElementIn/1 -> K1/1
  Sensor wP4r/1(w) -> Out Bus Element9/1
  Sensor wG2/1(w) -> Out Bus Element1/1
  Sensor wG3/1(w) -> Out Bus Element2/1
  Sensor wG4/1(w) -> Out Bus Element3/1
  Sensor wP4s/1(w) -> Out Bus Element8/1
  Sensor wP3r/1(w) -> Out Bus Element7/1
  Sensor wP2s/1(w) -> Out Bus Element6/1
  Sensor wP4c/1(w) -> Out Bus Element10/1
  BusElementIn7/1 -> Hydrostatic/1(Ctrl)
  BusElementIn8/1 -> HRB/1(str)
  Sensor P1s/1(w) -> Out Bus Element4/1
  Sensor wIn/1(w) -> Out Bus Element/1
  HRB/1(p) -> Out Bus Element12/1  "P_acc"
  Sensor wP1c/1(w) -> Out Bus Element5/1
  Sensor wOut/1(w) -> Out Bus Element11/1
  connections:
  Kr/RConn1 -- Gear Kr/LConn1
  Kv/RConn1 -- Gear Kv/RConn1
  Gears HS Out/RConn2 -- Sensor wG4/LConn1
  Gears HS Out/RConn1 -- Sensor P1s/LConn1
  Sensor wG3/LConn1 -- Power Sensor2 HS In/RConn1 -- Hydrostatic/LConn1
  Sensor wIn/LConn1 -- Power Sensor4c HRB/RConn1 -- HRB/RConn1
  Gears HS In/LConn2 -- Sensor wG2/LConn1
  Power Sensor6 CVT Out/LConn1 -- Inertia Out/LConn1
  Gear Kv/RConn2 -- Gear Kr/LConn2 -- Power Sensor7 BrkOut/LConn1 -- Sensor wOut/LConn1 -- Inertia Out/RConn1
  Planetary 3/LConn1 -- Sensor wP3r/LConn1
  Kb/LConn1 -- Mechanical Rotational Reference1/LConn1
  Kr/LConn1 -- Power Sensor7 BrkCarr/LConn1 -- Power Sensor5 PGOut/RConn1 -- Bearing Friction/LConn1 -- Sensor wP4c/LConn1 -- Kv/LConn1
  K4/RConn1 -- Planetary 4/LConn2 -- K3/RConn1
  K4/LConn1 -- Planetary 4/LConn3 -- K1/RConn1 -- K2/RConn1
  K1/LConn1 -- Planetary 3/RConn1
  K2/LConn1 -- Planetary 3/RConn3
  Planetary 3/LConn2 -- Planetary 2/RConn1
  Planetary 2/LConn2 -- Planetary 1/RConn1
  Planetary 1/RConn2 -- Planetary 2/LConn1 -- Sensor wP1c/LConn1
  Power Sensor1 CVT In/RConn1 -- Gears HS In/LConn1
  Planetary 2/RConn3 -- Planetary 3/LConn3 -- Sensor wP2s/LConn1
  K3/LConn1 -- Planetary 3/RConn2
  Kb/RConn1 -- Planetary 4/RConn1 -- Sensor wP4r/LConn1
  Power Sensor4a Sun1/LConn1 -- Gears HS Out/LConn1
  Planetary 4/RConn3 -- Sensor wP4s/LConn1
  Power Sensor1 CVT In/LConn1 -- E/RConn1
  Power Sensor2 HS In/LConn1 -- Gears HS In/RConn3
  Power Sensor3 HS Out/LConn1 -- Hydrostatic/RConn1
  Power Sensor4a Sun1/RConn1 -- Planetary 1/LConn3
  Gears HS In/RConn1 -- Power Sensor4b Ring1/LConn1
  Planetary 4/RConn2 -- Power Sensor5 PGOut/LConn1
  Power Sensor6 CVT Out/RConn1 -- D/RConn1
  Power Sensor3 HS Out/RConn1 -- Gears HS Out/LConn2
  Bearing Friction/RConn1 -- Mechanical Rotational Reference/LConn1
  Power Sensor4b Ring1/RConn1 -- Power Sensor4c HRB/LConn1 -- Planetary 1/LConn1
  Brake Carrier/RConn1 -- Power Sensor7 BrkCarr/RConn1
  Brake Out/RConn1 -- Power Sensor7 BrkOut/RConn1

== system sm_wheel_loader_lib/Controller ==
  vSpdCmd : Inport
  mCVT : Inport  Port=2
  mEngine : Inport  Port=3
  Bus Creator : BusCreator  Inputs=2
  Bus Selector : BusSelector  OutputSignals=ActuEngSpd(RPM),ActuEngTrq(Nm)
  CVT Ratio Ctrl : Subsystem
  Constant : Constant  Value=HMPST.Eng.wTarget
  Desired Ratio Calc : Subsystem
  Gain : Gain  Gain=pi/30/1000
  Product : Product
  Terminator : Terminator
  Transfer Fcn : TransferFcn  Denominator=[0.1 1]
  CVT : Outport
  Eng : Outport  Port=2
  wires:
  CVT Ratio Ctrl/1(CVT Ctrl) -> CVT/1
  Transfer Fcn/1 -> Desired Ratio Calc/1(CmdVehSpd (%))
  Bus Selector/1 -> Product/1, Desired Ratio Calc/2(ActuEngSpd (RPM))  "<ActuEngSpd(RPM)>"
  Desired Ratio Calc/1(Ratio (-)) -> CVT Ratio Ctrl/1(Ratio (-))  "Ratio (-)"
  Bus Selector/2 -> Product/2, Desired Ratio Calc/4(EngTrq (Nm))  "<ActuEngTrq(Nm)>"
  Product/1 -> Gain/1
  Gain/1 -> Terminator/1
  mCVT/1 -> Desired Ratio Calc/3(CVTFeedback)
  Desired Ratio Calc/3(HRBCtrl (-)) -> CVT Ratio Ctrl/3(HRBCtrl (-))
  Desired Ratio Calc/5(CmdSpdRate) -> Bus Creator/1  "CmdSpdRate"
  Constant/1 -> Bus Creator/2  "CmdEngSpd(RPM)"
  Bus Creator/1 -> Eng/1
  mEngine/1 -> Bus Selector/1
  Desired Ratio Calc/4(MBCtrl (-)) -> CVT Ratio Ctrl/4(MBCtrl (-))
  Desired Ratio Calc/2(CmdVehSpdDir) -> CVT Ratio Ctrl/2(CmdVehSpdDir)
  vSpdCmd/1 -> Transfer Fcn/1

== system sm_wheel_loader_lib/Engine Droop ==
  EngCtrl : Inport
  Bus Creator : BusCreator  Inputs=2
  Bus Selector : BusSelector  OutputSignals=CmdEngSpd(RPM)
  Bus Selector1 : BusSelector  OutputSignals=tEngMax
  Constant : Constant  Value=0.2
  Engine Management : engine_mgmt_lib/Engine Management  kp_thr=10  ki_thr=0  kp_brk=5  ki_brk=0  engine_trq=HMPST.Eng.MaxTorq.TrqVec  engine_spd=HMPST.Eng.MaxTorq.SpdVec  w0_engine=HMPST.Eng.wTarget
  Generic Engine : sdl_lib/Engines & Motors/Generic Engine  input_type=sdl.enum.GenericEngineInputType.NormalizedThrottle  model_parameterization=sdl.enum.engineParameterization.torque  engine_type=sdl.enum.engineType.SI  Trq_max=380 N*m  w_Trq_max=4300 rpm  P_max=230 kW  w_P_max=6858 rpm  w_max=7000 rpm  w_min=500 rpm  w_tab=[HMPST.Eng.MaxTorq.SpdVec(2:end) 3000] rpm  trq_tab=[HMPST.Eng.MaxTorq.TrqVec(2:end-2) 10 10 10] N*m  pwr_tab=[10, 30, 70, 110, 165, 190, 220, 230] kW  interp_method=simscape.enum.interpolation.linear  w_thr=100 rpm  model_inertia=sdl.enum.model_inertia.on  inertia=1 kg*m^2  initial_velocity=HMPST.Eng.wTarget rpm  model_time_constant=sdl.enum.lagOffOn.off  time_constant=0.2 s  initial_normalized_throttle=0  fc_model=sdl.enum.fuel_consumption_model.FuelOff  fc_per_rev=25 mg/rev  fc_w_tab=[1000, 2000, 3000, 4000, 5000, 6000] rpm  fc_trq_tab=[0, 80, 160, 200, 240, 320, 360, 400] N*m  fc_tab=[.5, .9, 1.4, 1.6, 1.9, 2.7, 3.4, 4.4; 1, 1.7, 2.7, 3.1, 3.6, 5, 6, 7.4; 1.4, 2.7, 4, 4.8, 5.6, 7.5, 8.5, 10.5; 2, 3.6, 5.8, 6.7, 8, 10.4, 11.7, 13.3; 2.5, 4.8, 7.9, 9.4, 10.8, 14, 16.2, 18.6; 3.1, 6, 10.3, 11.9, 13.8, 18.4, 22, 26.5] g/s  bmep_tab=[0, 250, 500, 625, 750, 1000, 1150, 1250] kPa  bsfc_tab=[410, 380, 300, 280, 270, 290, 320, 380; 410, 370, 290, 270, 260, 270, 285, 320; 415, 380, 290, 275, 265, 270, 270, 300; 420, 390, 310, 290, 285, 280, 280, 285; 430, 410, 340, 320, 310, 300, 310, 320; 450, 430, 370, 340, 330, 330, 350, 380] g/(hr*kW)  fc_interp_method=simscape.enum.interpolation.linear  displaced_volume=400 cm^3  rev_per_cycle=2  idle_speed=false  idle_speed_reference=1000 rpm  tau_controller=1 s  idle_w_thr=1 rpm  redline=false  redline_speed=5000 rpm  tau_redline=1 s  redline_w_thr=1 rpm
      settings: InternalSimscapePortConfiguration="{\"Bottom\":[],\"Left\":[{\"id\":\"ThrNorm\",\"label\":\"Thr\",\"type\":\"input\"},{\"id\":\"B\",\"label\":\"B\",\"type\":\"foundation.mechanical.rotational.rotational\"}],\"Right\":[{\"id\":\"P\",\"label\":\"P\",\"type\":\"output\"},{\"id\":\"FC\",\"label\":\"FC\",\"type\":\"output\"},{\"id\":\"F\",\"label\":\"F\",\"type\":\"foundation.mechanical.rotational.rotational\"}],\"Top\":[]}"
  Mechanical Rotational Reference : fl_lib/Mechanical/Rotational Elements/Mechanical Rotational Reference
  Simulink-PS Converter : nesl_utility/Simulink-PS Converter  PhysicalDomain=network_engine_domain  SubClassName=ps_input  LeftPortType=input  RightPortType=output  PseudoPeriodic=off  Frequencies=[]  NoiseDistribution=none  NoiseParameters=[]  Unit=1  AffineConversion=off  FilteringAndDerivatives=provide  SimscapeFilterOrder=1  InputFilterTimeConstant=0.001  UdotUserProvided=0
  Speed Sensor : Subsystem
  Terminator1 : Terminator
  Torque Sensor : Subsystem
      settings: PortSchema="{\"entries\":[{\"content\":{\"sides\":[{\"content\":{\"connectorIds\":[\"LConn1\"]},\"type\":\"ConnectorPlacement.EquallySpacedRectSide\",\"uuid\":\"5a764f16-cafe-4867-b916-6b4e7e02daa5\"},{\"content\":{\"connectorIds\":[\"RConn1\"],\"side\":\"RIGHT\"},\"type\":\"ConnectorPlacement.EquallySpacedRectSide\",\"uuid\":\"8ceee8ac-f09f-4a1d-836f-79964ce3b2d4\"},{\"content\":{\"connectorIds\":[\"Out1\"],\"side\":\"TOP\"},\"type\":\"ConnectorPlacement.EquallySpacedRectSide\",\"uuid\":\"effcec0c-0a3a-409b-822c-5f5bf6cd9579\"}]},\"type\":\"ConnectorPlacement.EquallySpacedConnector\",\"uuid\":\"cbc631ce-3260-4296-836f-4219c3ba8d3a\"}],\"packageUris\":[\"http://schema.mathworks.com/mf0/Connector/R2020b\"],\"version\":\"1.0\"}"
  Shaft : PMIOPort  Side=Right
  EngFbk : Outport
  Out Bus Element : Outport  Port=2  PortName=m  Element=w.cmd
  Out Bus Element1 : Outport  Port=2  PortName=m  Element=w.meas
  Out Bus Element2 : Outport  Port=2  PortName=m  Element=trq.limUp
  Out Bus Element3 : Outport  Port=2  PortName=m  Element=trq.meas
  Out Bus Element4 : Outport  Port=2  PortName=m  Element=trq.Cmd
  wires:
  Torque Sensor/1(m) -> Out Bus Element3/1
  Engine Management/1 -> Simulink-PS Converter/1  "Throttle"
  Bus Creator/1 -> EngFbk/1
  EngCtrl/1 -> Bus Selector/1
  Speed Sensor/1(rpm) -> Engine Management/1, Out Bus Element1/1, Bus Creator/2  "ActuEngSpd(RPM)"
  Bus Selector1/1 -> Out Bus Element2/1  "<tEngMax>"
  Engine Management/4 -> Bus Creator/1, Out Bus Element4/1  "ActuEngTrq(Nm)"
  Bus Selector/1 -> Out Bus Element/1, Engine Management/2  "<CmdEngSpd(RPM)>"
  Constant/1 -> Engine Management/3
  Engine Management/3 -> Bus Selector1/1
  Engine Management/2 -> Terminator1/1
  connections:
  Simulink-PS Converter/RConn1 -- Generic Engine/LConn1
  Speed Sensor/LConn1 -- Torque Sensor/LConn1 -- Generic Engine/RConn3
  Mechanical Rotational Reference/LConn1 -- Generic Engine/LConn2
  Shaft/RConn1 -- Torque Sensor/RConn1
